simulink model "elmak"  (R2023b)
settings: Solver=VariableStepAuto  StartTime=0.0  StopTime=5.0  RelTol=1e-3
libraries: spsControlledVoltageSourceLib x2, spsVoltageMeasurementLib x2, spsDCMachineLib x1, sps_lib x1
settings Model: Creator=Muhammed Kılıç  LastModifiedBy=CASPER

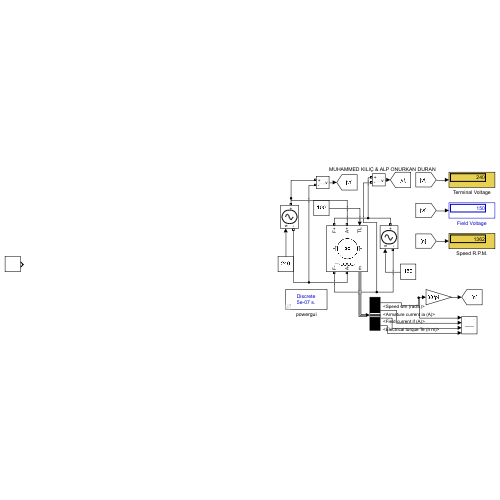
[thumbnail: Simulink's stored preview of the top-level diagram]
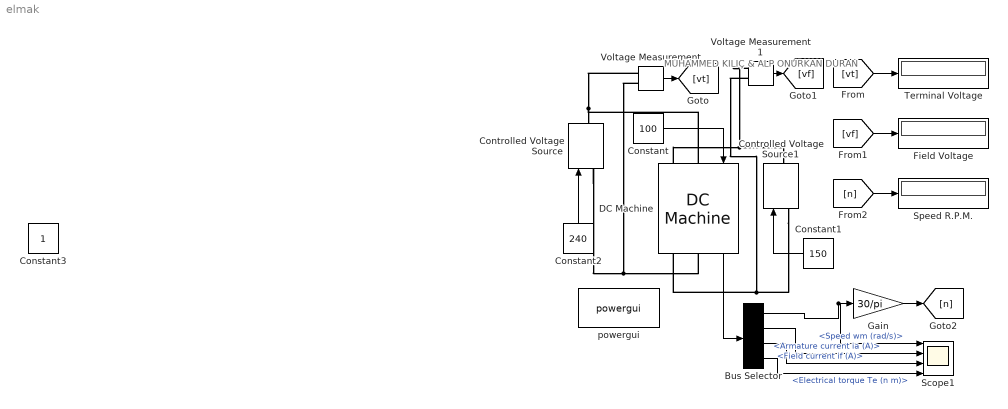
== system elmak ==
  note: MUHAMMED KILIÇ & ALP ONURKAN DURAN
  Bus Selector : BusSelector  OutputSignals=Speed wm (rad/s),Armature current ia (A),Field current if (A),Electrical torque Te (n m)
  Constant : Constant  Value=100
  Constant1 : Constant  Value=150
  Constant2 : Constant  Value=240
  Constant3 : Constant
  Controlled Voltage Source : spsControlledVoltageSourceLib/Controlled Voltage Source  Initialize=on  Source_Type=AC  Amplitude=0  Phase=0  Frequency=0  Measurements=None
  Controlled Voltage Source1 : spsControlledVoltageSourceLib/Controlled Voltage Source  Initialize=on  Source_Type=AC  Amplitude=0  Phase=0  Frequency=0  Measurements=None
  DC Machine : spsDCMachineLib/DC Machine  PresetModel=No  MechanicalLoad=Torque TL  FieldType=Wound  ShowDetailedParameters=on  MeasurementBus=off  RLa=[0.78 0.016]  RLf=[150 112.5]  Laf=1.234  MachineConstant=Torque constant (N.m/A)  Ke=1.8  Kt=1.8  J=0.05  Bm=0.01  Tf=0  w0=1  Ifinit=0  TsPowergui=0  TsBlock=-1
  Field Voltage : Display
  Gain : Gain  Gain=30/pi
  Scope1 : Scope  NumInputPorts=4
  Speed R.P.M. : Display
  Terminal Voltage : Display
  Voltage Measurement : spsVoltageMeasurementLib/Voltage Measurement  PhasorSimulation=off  OutputType=Complex  PSBequivalent=0
  Voltage Measurement1 : spsVoltageMeasurementLib/Voltage Measurement  PhasorSimulation=off  OutputType=Complex  PSBequivalent=0
  powergui : sps_lib/powergui  Priority=1  SimulationMode=Discrete  SampleTime=5e-7  frequency=60  Iterations=50  frequencyindice=0  Pbase=100e6  ErrMax=1e-4  UnitsV=kV  UnitsW=MW  buscounter=0  FunctionMessages=off  echomessages=off  EnableUseOfTLC=off  CurrentSourceSwitches=off  DisableSnubberDevices=off  DisableRonSwitches=off  DisableVfSwitches=off  DisplayEquations=off  AutomaticDiscreteSolvers=off  SolverType=Tustin/Backward Euler (TBE)  Interpol=off  ExternalGateDelay=off  methode=off  Ts=100  x0status=blocks  SPID=on  SwTol=0  HookPort=off  NonlinearTolerance=1e-4  nMaxIteration=100  ContinueOnMaxIteration=off  RestoreLinks=warning  ResistiveCurrentMeasurement=off  Frange=[0:2:500]  Ylog=off  Xlog=on  ShowGrid=off  save=off  variable=ZData  structure=0  ZoomFFT=off  StartTime=0.0  cycles=1  DisplayStyle=1  fundamental=60  FreqAxis=off  MaxFrequency=1000  frequencyindicesteady=1  RmsSteady=1  display=off
  wires:
  Constant2/1 -> Controlled Voltage Source/1
  Constant/1 -> DC Machine/1
  Constant1/1 -> Controlled Voltage Source1/1
  Voltage Measurement1/1 -> [vf]
  DC Machine/1 -> Bus Selector/1
  Gain/1 -> [n]
  [vf] -> Field Voltage/1
  [n] -> Speed R.P.M./1
  [vt] -> Terminal Voltage/1
  Bus Selector/1 -> Scope1/1, Gain/1  "<Speed wm (rad/s)>"
  Bus Selector/2 -> Scope1/2  "<Armature current ia (A)>"
  Bus Selector/3 -> Scope1/3  "<Field current if (A)>"
  Bus Selector/4 -> Scope1/4  "<Electrical torque Te (n m)>"
  Voltage Measurement/1 -> [vt]
  connections:
  DC Machine/LConn1 -- Voltage Measurement/LConn1 -- Controlled Voltage Source/RConn1
  Controlled Voltage Source/LConn1 -- Voltage Measurement/LConn2 -- DC Machine/RConn1
  DC Machine/LConn2 -- Voltage Measurement1/LConn1 -- Controlled Voltage Source1/RConn1
  Controlled Voltage Source1/LConn1 -- Voltage Measurement1/LConn2 -- DC Machine/RConn2
